simulink model "ADRC_2nd_Order_Kang"  (R2024b)
settings: Solver=FixedStepAuto  StartTime=0.0  StopTime=20  FixedStep=0.01  RelTol=1e-3
values from neighbouring files (symbols this model uses):
  a = p.x_model(1)    [Run_MPC_For_2nd_order_Plant.m]    (also in Run_MPC_For_2nd_order_Plant_auto_tuning.m = x_model(1))
  b = p.x_model(3)    [Run_MPC_For_2nd_order_Plant.m]    (also in Run_MPC_For_2nd_order_Plant_auto_tuning.m = x_model(3))
  c = p.x_model(2)    [Run_MPC_For_2nd_order_Plant.m]    (also in Run_MPC_For_2nd_order_Plant_auto_tuning.m = x_model(2))
  f0 = p.x_model(4)    [Run_MPC_For_2nd_order_Plant.m]    (also in Run_MPC_For_2nd_order_Plant_auto_tuning.m = x_model(4))
  T_sample = .01    (= 0.01)    [Run_MPC_For_2nd_order_Plant.m]    (also in Run_MPC_For_2nd_order_Plant_auto_tuning.m)
settings Model: Creator=HUAWEI  LastModifiedBy=sk3547969879
settings ModelReferenceCC: EnableRefExpFcnMdlSchedulingChecks=on
settings RTWCC: GPUComputeCapability=3.5

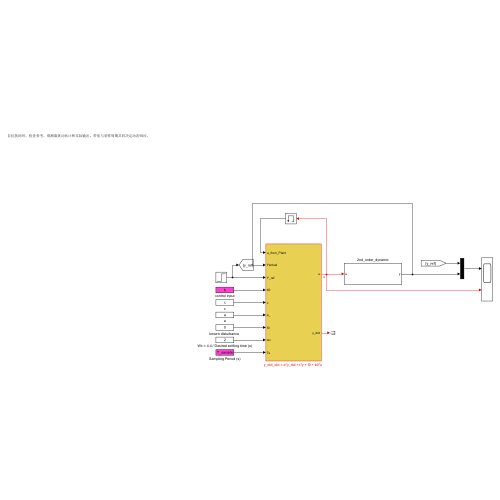
[thumbnail: Simulink's stored preview of the top-level diagram]
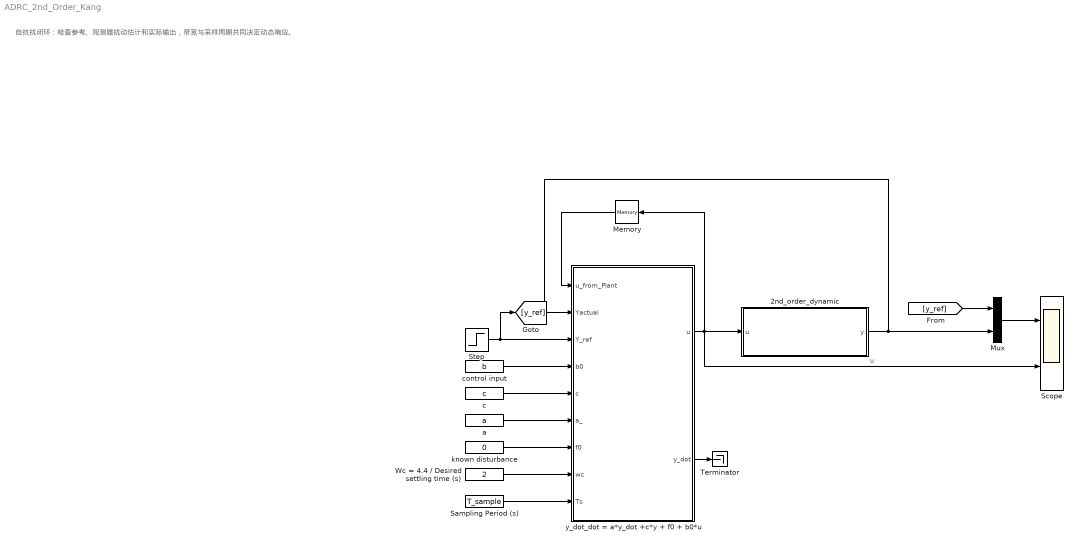
== system ADRC_2nd_Order_Kang ==
  note: 自抗扰闭环：检查参考、观测器扰动估计和实际输出，带宽与采样周期共同决定动态响应。
  2nd_order_dynamic : Subsystem
  Memory : Memory
  Mux : Mux  Inputs=2
  Sampling Period (s) : Constant  Value=T_sample
  Scope : Scope  NumInputPorts=2
  Step : Step  Time=5  SampleTime=0
  Terminator : Terminator
  Wc = 4.4 / Desired settling time (s) : Constant  Value=2
  a : Constant  Value=a
  c : Constant  Value=c
  control input : Constant  Value=b
  "known disturbance " : Constant  Value=0
  "y_dot_dot = a*y_dot +c*y + f0 + b0*u " : Subsystem
  wires:
  a/1 -> "y_dot_dot = a*y_dot +c*y + f0 + b0*u "/6(a_)
  c/1 -> "y_dot_dot = a*y_dot +c*y + f0 + b0*u "/5(c)
  control input/1 -> "y_dot_dot = a*y_dot +c*y + f0 + b0*u "/4(b0)
  "y_dot_dot = a*y_dot +c*y + f0 + b0*u "/1(u) -> 2nd_order_dynamic/1(u), Memory/1, Scope/2  "u"
  Memory/1 -> "y_dot_dot = a*y_dot +c*y + f0 + b0*u "/1(u_from_Plant)
  2nd_order_dynamic/1(y) -> "y_dot_dot = a*y_dot +c*y + f0 + b0*u "/2(Yactual), Mux/2
  Step/1 -> [y_ref], "y_dot_dot = a*y_dot +c*y + f0 + b0*u "/3(Y_ref)
  Wc = 4.4 / Desired settling time (s)/1 -> "y_dot_dot = a*y_dot +c*y + f0 + b0*u "/8(wc)
  Sampling Period (s)/1 -> "y_dot_dot = a*y_dot +c*y + f0 + b0*u "/9(Ts)
  "known disturbance "/1 -> "y_dot_dot = a*y_dot +c*y + f0 + b0*u "/7(f0)
  [y_ref] -> Mux/1
  Mux/1 -> Scope/1
  "y_dot_dot = a*y_dot +c*y + f0 + b0*u "/2(y_dot) -> Terminator/1

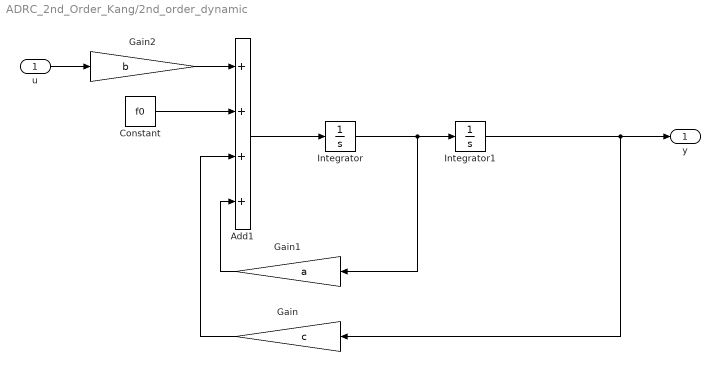
== system ADRC_2nd_Order_Kang/2nd_order_dynamic ==
  u : Inport
  Add1 : Sum  Inputs=++++
  Constant : Constant  Value=f0
  Gain : Gain  Gain=c
  Gain1 : Gain  Gain=a
  Gain2 : Gain  Gain=b
  Integrator : Integrator
  Integrator1 : Integrator
  y : Outport
  wires:
  Add1/1 -> Integrator/1
  Gain/1 -> Add1/3
  u/1 -> Gain2/1
  Integrator/1 -> Gain1/1, Integrator1/1
  Integrator1/1 -> Gain/1, y/1
  Gain2/1 -> Add1/1
  Gain1/1 -> Add1/4
  Constant/1 -> Add1/2

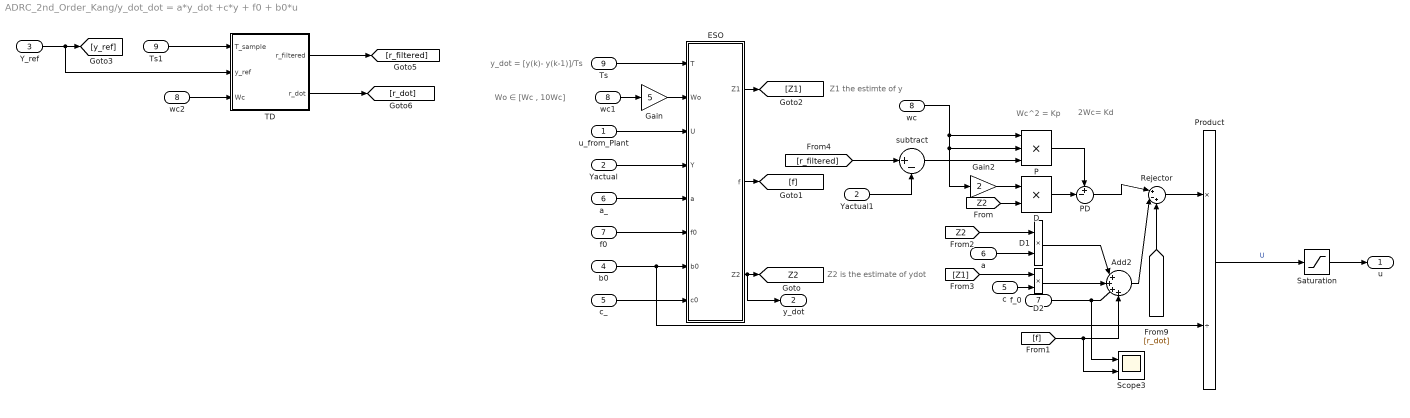
== system ADRC_2nd_Order_Kang/y_dot_dot = a*y_dot +c*y + f0 + b0*u  ==
  note: 2Wc= Kd
  note: Wc^2 = Kp
  note: Z2 is the estimate of ydot
  note: Z1 the estimte of y
  note: Wo ∈ [Wc , 10Wc]
  note: y_dot = [y(k)- y(k-1)]/Ts
  u_from_Plant : Inport
  Yactual : Inport  Port=2
  Y_ref : Inport  Port=3
  b0 : Inport  Port=4
  c : Inport  Port=5
  a_ : Inport  Port=6
  f0 : Inport  Port=7
  wc : Inport  Port=8
  Ts : Inport  Port=9
  Add2 : Sum  Inputs=|++++
  D : Product  RndMeth=Zero
  D1 : Product  RndMeth=Zero
  D2 : Product  RndMeth=Zero
  ESO : Subsystem
  Gain : Gain  Gain=5
  Gain2 : Gain  Gain=2
  P : Product  Inputs=3  RndMeth=Zero
  PD : Sum  Inputs=+-|
  Product : Product  Inputs=*/  RndMeth=Zero
  Rejector : Sum  Inputs=|+-+
  Saturation : Saturate  UpperLimit=inf  LowerLimit=-inf
  Scope3 : Scope  NumInputPorts=2
  TD : Subsystem
  Ts1 : InportShadow  Port=9
  Yactual1 : InportShadow  Port=2
  a : InportShadow  Port=6
  c_ : InportShadow  Port=5
  f_0 : InportShadow  Port=7
  subtract : Sum  Inputs=|+-
  wc1 : InportShadow  Port=8
  wc2 : InportShadow  Port=8
  u : Outport  VectorParamsAs1DForOutWhenUnconnected=off
  y_dot : Outport  Port=2  VectorParamsAs1DForOutWhenUnconnected=off
  tag scope: Z2=global
  wires:
  [Z2] -> D1/1
  a/1 -> D1/2
  D1/1 -> Add2/1
  Ts/1 -> ESO/1(T)
  wc1/1 -> Gain/1
  u_from_Plant/1 -> ESO/3(U)
  Yactual/1 -> ESO/4(Y)
  a_/1 -> ESO/5(a)
  f0/1 -> ESO/6(f0)
  ESO/2(f) -> [f]
  [Z2] -> D/2
  b0/1 -> Product/2, ESO/7(b0)
  Product/1 -> Saturation/1  "U"
  subtract/1 -> P/3
  Gain2/1 -> D/1
  wc/1 -> Gain2/1, P/2, P/1
  P/1 -> PD/1
  ESO/3(Z2) -> y_dot/1, [Z2]
  D/1 -> PD/2
  PD/1 -> Rejector/1
  f_0/1 -> Scope3/1, Add2/3
  [f] -> Scope3/2, Add2/4
  Add2/1 -> Rejector/2
  Rejector/1 -> Product/1
  c_/1 -> ESO/8(c0)
  c/1 -> D2/2
  Yactual1/1 -> subtract/2
  D2/1 -> Add2/2
  ESO/1(Z1) -> [Z1]
  [Z1] -> D2/1
  Gain/1 -> ESO/2(Wo)
  [r_dot] -> Rejector/3
  Saturation/1 -> u/1
  [r_filtered] -> subtract/1
  Ts1/1 -> TD/1(T_sample)
  Y_ref/1 -> TD/2(y_ref), [y_ref]
  TD/1(r_filtered) -> [r_filtered]
  TD/2(r_dot) -> [r_dot]
  wc2/1 -> TD/3(Wc)

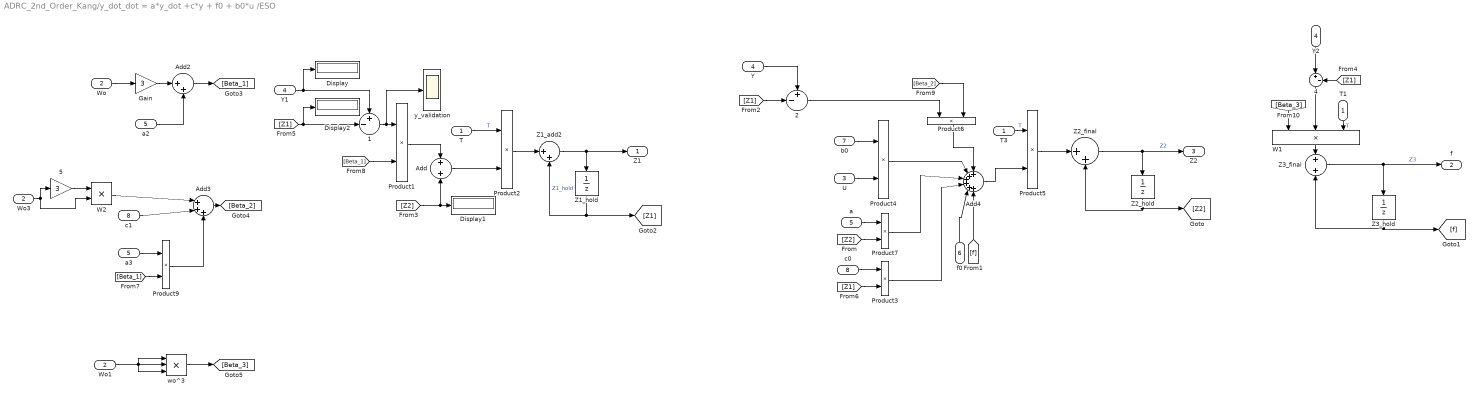
== system ADRC_2nd_Order_Kang/y_dot_dot = a*y_dot +c*y + f0 + b0*u /ESO ==
  T : Inport
  Wo : Inport  Port=2
  U : Inport  Port=3
  Y : Inport  Port=4
  a : Inport  Port=5
  f0 : Inport  Port=6
  b0 : Inport  Port=7
  c0 : Inport  Port=8
  1 : Sum  Inputs=+-|
  2 : Sum  Inputs=+-|
  4 : Sum  Inputs=|+-
  5 : Gain  Gain=3
  Add : Sum
  Add2 : Sum  Inputs=|++
  Add3 : Sum  Inputs=|+++
  Add4 : Sum  Inputs=++++++
  Display : Display
  Display1 : Display
  Display2 : Display
  Gain : Gain  Gain=3
  Product{1..7,9} (8 alike) : Product  RndMeth=Zero
  T1 : InportShadow
  T3 : InportShadow
  W1 : Product  Inputs=3  RndMeth=Zero
  W2 : Product  RndMeth=Zero
  Wo1 : InportShadow  Port=2
  Wo3 : InportShadow  Port=2
  Y1 : InportShadow  Port=4
  Y2 : InportShadow  Port=4
  Z1_add2 : Sum  Inputs=|++
  Z1_hold : UnitDelay  SampleTime=-1  HasFrameUpgradeWarning=on
  Z2_final : Sum  Inputs=|++
  Z2_hold : UnitDelay  SampleTime=-1  HasFrameUpgradeWarning=on
  Z3_final : Sum
  Z3_hold : UnitDelay  SampleTime=-1  HasFrameUpgradeWarning=on
  a2 : InportShadow  Port=5
  a3 : InportShadow  Port=5
  c1 : InportShadow  Port=8
  wo^3 : Product  Inputs=3  RndMeth=Zero
  y_validation : Scope
  Z1 : Outport  VectorParamsAs1DForOutWhenUnconnected=off
  f : Outport  Port=2  VectorParamsAs1DForOutWhenUnconnected=off
  Z2 : Outport  Port=3  VectorParamsAs1DForOutWhenUnconnected=off
  wires:
  Z3_hold/1 -> [f], Z3_final/2
  f0/1 -> Add4/5
  Y1/1 -> Display/1, 1/1
  [Z1] -> Display2/1, 1/2
  Wo1/1 -> wo^3/1, wo^3/2, wo^3/3
  [Z1] -> 4/2
  Y2/1 -> 4/1
  4/1 -> W1/2
  [Z2] -> Add/2, Display1/1
  Y/1 -> 2/1
  [Z1] -> 2/2
  [Z2] -> Product7/2
  T3/1 -> Product5/1  "T"
  T1/1 -> W1/3  "T"
  Product7/1 -> Add4/3
  a/1 -> Product7/1
  Product6/1 -> Add4/1
  [Beta_1] -> Product1/2
  1/1 -> y_validation/1, Product1/1
  Product1/1 -> Add/1
  T/1 -> Product2/1  "T"
  Add/1 -> Product2/2
  Product2/1 -> Z1_add2/1
  Z1_add2/1 -> Z1_hold/1, Z1/1
  Product4/1 -> Add4/2
  2/1 -> Product6/1
  Add4/1 -> Product5/2
  Product5/1 -> Z2_final/1
  [Beta_3] -> W1/1
  W1/1 -> Z3_final/1
  Z2_final/1 -> Z2/1, Z2_hold/1  "Z2"
  U/1 -> Product4/2
  Z1_hold/1 -> Z1_add2/2, [Z1]  "Z1_hold"
  Z2_hold/1 -> [Z2], Z2_final/2
  Z3_final/1 -> Z3_hold/1, f/1  "Z3"
  b0/1 -> Product4/1
  Wo/1 -> Gain/1
  Product3/1 -> Add4/4
  [Z1] -> Product3/2
  c0/1 -> Product3/1
  wo^3/1 -> [Beta_3]
  Gain/1 -> Add2/1
  Add2/1 -> [Beta_1]
  a2/1 -> Add2/2
  Wo3/1 -> 5/1, W2/2
  5/1 -> W2/1
  W2/1 -> Add3/1
  c1/1 -> Add3/2
  a3/1 -> Product9/1
  Add3/1 -> [Beta_2]
  [Beta_1] -> Product9/2
  Product9/1 -> Add3/3
  [Beta_2] -> Product6/2
  [f] -> Add4/6

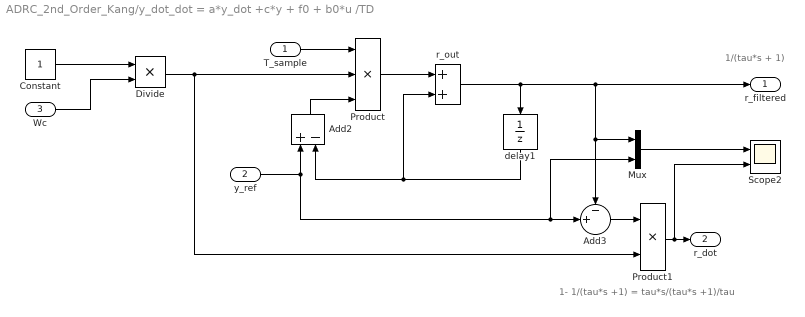
== system ADRC_2nd_Order_Kang/y_dot_dot = a*y_dot +c*y + f0 + b0*u /TD ==
  note: 1- 1/(tau*s +1) = tau*s/(tau*s +1)/tau
  note: 1/(tau*s + 1)
  T_sample : Inport
  y_ref : Inport  Port=2
  Wc : Inport  Port=3
  Add2 : Sum  Inputs=+-
  Add3 : Sum  Inputs=-+|
  Constant : Constant
  Divide : Product  Inputs=**
  Mux : Mux  Inputs=2
  Product : Product  Inputs=3  RndMeth=Zero
  Product1 : Product  RndMeth=Zero
  Scope2 : Scope  NumInputPorts=2
  delay1 : UnitDelay  SampleTime=-1  HasFrameUpgradeWarning=on
  r_out : Sum
  r_filtered : Outport  VectorParamsAs1DForOutWhenUnconnected=off
  r_dot : Outport  Port=2  VectorParamsAs1DForOutWhenUnconnected=off
  wires:
  T_sample/1 -> Product/1
  Divide/1 -> Product/2, Product1/2
  Add3/1 -> Product1/1
  r_out/1 -> r_filtered/1, Mux/1, Add3/1, delay1/1
  Add2/1 -> Product/3
  Product1/1 -> Scope2/2, r_dot/1
  delay1/1 -> r_out/2, Add2/2
  y_ref/1 -> Mux/2, Add3/2, Add2/1
  Product/1 -> r_out/1
  Mux/1 -> Scope2/1
  Constant/1 -> Divide/1
  Wc/1 -> Divide/2
